simulink model "day28_closed_loop_vehicle_control"  (R2026a)
settings: Solver=VariableStepAuto
settings Model: Creator=hem23  LastModifiedBy=hem23

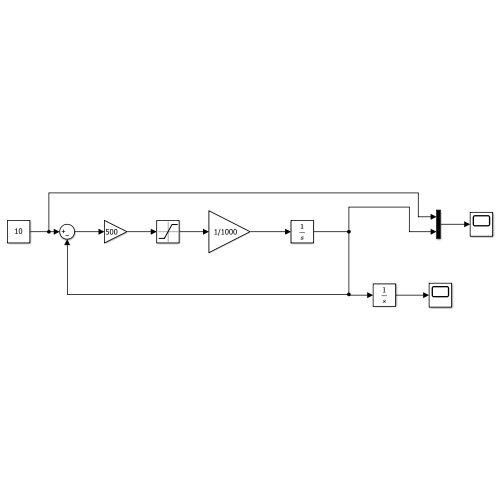
[thumbnail: Simulink's stored preview of the top-level diagram]
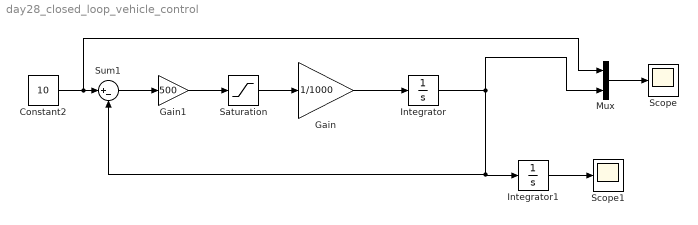
== system day28_closed_loop_vehicle_control ==
  Constant2 : Constant  Value=10
  Gain : Gain  Gain=1/1000
  Gain1 : Gain  Gain=500
  Integrator : Integrator
  Integrator1 : Integrator
  Mux : Mux  Inputs=2
  Saturation : Saturate  UpperLimit=2000  LowerLimit=0
  Scope : Scope
      settings: ActiveDisplayYMinimum=-1.2499999999999998  ActiveDisplayYMaximum=11.25
  Scope1 : Scope
      settings: ActiveDisplayYMinimum=-11.419120974803699  ActiveDisplayYMaximum=96.824109799753217
  Sum1 : Sum  Inputs=|+-
  wires:
  Gain/1 -> Integrator/1
  Integrator/1 -> Sum1/2, Integrator1/1, Mux/2
  Mux/1 -> Scope/1
  Constant2/1 -> Mux/1, Sum1/1
  Sum1/1 -> Gain1/1
  Gain1/1 -> Saturation/1
  Saturation/1 -> Gain/1
  Integrator1/1 -> Scope1/1
